simulink model "TransformerB_v4"  (R2023a)
settings: Solver=ode23tb  StartTime=0.0  StopTime=1  MaxStep=1e-4  RelTol=1e-3  EnableMultiTasking=on
undefined symbols (not defined in the file or in its folder): D11, Delta
libraries: spsSeriesRLCBranchLib x18, spsGroundLib x9, spsSaturableTransformerLib x6, spsCurrentMeasurementLib x6, spsThreePhaseFaultLib x6, spsRMSLib x6, dspstat3 x5, spsACVoltageSourceLib x3, spsThreePhaseVIMeasurementLib x2, spsThreePhaseBreakerLib x2, simulink_extras x1, simulink x1
settings Model: Creator=Admin  LastModifiedBy=Abeer
settings DataIOCC: LimitDataPoints=on  SaveFormat=Array
settings OptimizationCC: LifeSpan=inf
settings DebuggingCC: AlgebraicLoopMsg=none  SolverPrmCheckMsg=warning  SFUnexpectedBacktrackingDiag=warning  SFNoUnconditionalDefaultTransitionDiag=warning  SFExecutionAtInitializationDiag=none  ArithmeticOperatorsInVariantConditions=warning
settings HardwareCC: ProdBitPerPointer=32  ProdBitPerSizeT=32  ProdBitPerPtrDiffT=32  ProdLargestAtomicFloat=None  ProdIntDivRoundTo=Undefined  ProdEndianess=Unspecified  ProdWordSize=32  ProdHWDeviceType=32-bit Generic
settings ModelReferenceCC: PropagateSignalLabelsOutOfModel=off
settings SFSimCC: SimUseLocalCustomCode=off  CustomCodeUndefinedFunction=UseInterfaceOnly
settings RTWCC: RTWUseLocalCustomCode=off
settings CodeAppCC: StateflowObjectComments=on
settings GRTTargetCC: TargetLangStandard=C89/C90 (ANSI)
settings ConfigComp: CovMetricSettings=dw  CovSaveCumulativeToWorkspaceVar=on  CovSaveSingleToWorkspaceVar=on  CovExternalEMLEnable=off  CovSFcnEnable=off
settings SimscapeCC: SimscapeNormalizeSystem=off

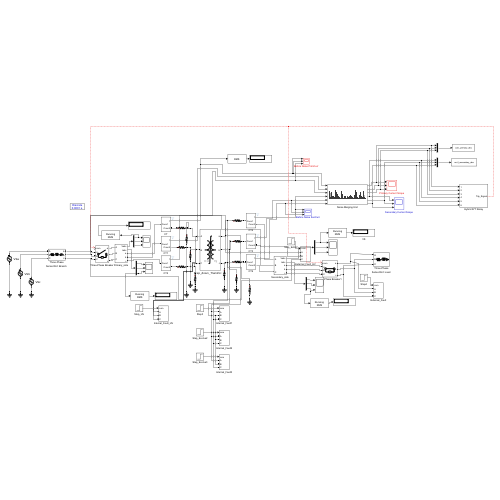
[thumbnail: Simulink's stored preview of the top-level diagram]
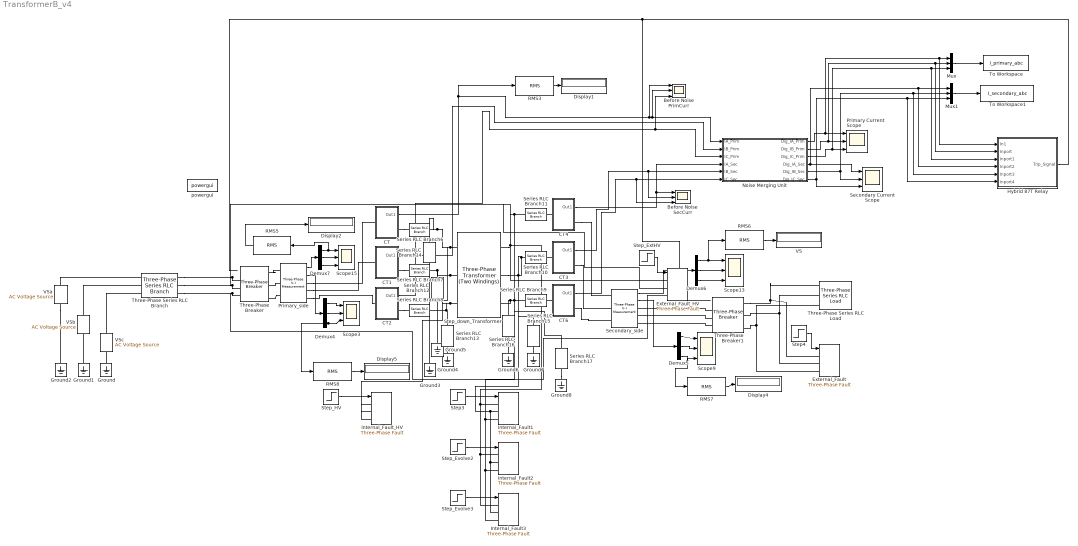
== system TransformerB_v4 ==
  Before Noise PrimCurr : Scope  NumInputPorts=3
  Before Noise SecCurr : Scope  NumInputPorts=3
  CT : Subsystem
  CT1 : Subsystem
  CT2 : Subsystem
  CT3 : Subsystem
  CT4 : Subsystem
  CT6 : Subsystem
  Demux{4..7} (4 alike) : Demux  Outputs=3
  Display{1..2,4..5} (4 alike) : Display
  External_Fault : spsThreePhaseFaultLib/Three-Phase Fault  InitialStates=0  FaultA=off  FaultB=off  FaultC=off  GroundFault=off  SwitchTimes=[0.05 1]  External=on  SwitchStatus=NaN  FaultResistance=0.001  GroundResistance=0.001  SnubberResistance=1e6  SnubberCapacitance=inf  Measurements=None
  External_Fault_HV : spsThreePhaseFaultLib/Three-Phase Fault  InitialStates=0  FaultA=off  FaultB=off  FaultC=off  GroundFault=off  SwitchTimes=[0.05 1]  External=on  SwitchStatus=NaN  FaultResistance=0.01  GroundResistance=0.01  SnubberResistance=1e6  SnubberCapacitance=inf  Measurements=None
  Ground{,1..8} (9 alike) : spsGroundLib/Ground  LConnTagsString=a
  Hybrid 87T Relay : Subsystem
  Internal_Fault1 : spsThreePhaseFaultLib/Three-Phase Fault  InitialStates=0  FaultA=off  FaultB=off  FaultC=off  GroundFault=off  SwitchTimes=[0.05 1]  External=on  SwitchStatus=NaN  FaultResistance=0.1  GroundResistance=0.01  SnubberResistance=1e6  SnubberCapacitance=inf  Measurements=None
  Internal_Fault2 : spsThreePhaseFaultLib/Three-Phase Fault  InitialStates=0  FaultA=off  FaultB=off  FaultC=off  GroundFault=off  SwitchTimes=[0.05 1]  External=on  SwitchStatus=NaN  FaultResistance=0.01  GroundResistance=0.01  SnubberResistance=1e6  SnubberCapacitance=inf  Measurements=None
  Internal_Fault3 : spsThreePhaseFaultLib/Three-Phase Fault  InitialStates=0  FaultA=off  FaultB=off  FaultC=off  GroundFault=off  SwitchTimes=[0.05 1]  External=on  SwitchStatus=NaN  FaultResistance=0.01  GroundResistance=0.01  SnubberResistance=1e6  SnubberCapacitance=inf  Measurements=None
  Internal_Fault_HV : spsThreePhaseFaultLib/Three-Phase Fault  InitialStates=0  FaultA=off  FaultB=off  FaultC=off  GroundFault=off  SwitchTimes=[0.05 1]  External=on  SwitchStatus=NaN  FaultResistance=0.01  GroundResistance=0.01  SnubberResistance=1e6  SnubberCapacitance=inf  Measurements=None
  Mux : Mux  Inputs=3
  Mux1 : Mux  Inputs=3
  Noise Merging Unit : Subsystem
      mask Display: image('$imagefile'); % Use "Edit Image" on toolstrip to change.
  Primary Current Scope : Scope  NumInputPorts=3
  Primary_side : spsThreePhaseVIMeasurementLib/Three-Phase V-I Measurement  VoltageMeasurement=phase-to-phase  SetLabelV=off  LabelV=Vabc  Vpu=off  VpuLL=off  CurrentMeasurement=yes  SetLabelI=off  LabelI=Iabc  Ipu=off  Pbase=100e6  Vbase=500e3  OutputType=Complex  PhasorSimulation=off  PSBequivalent=0
  RMS3 : dspstat3/RMS  run=off  directionMode=Each column  dimension=1  InputProcessing=Columns as channels (frame based)  reset_popup=None
  RMS{5..8} (4 alike) : dspstat3/RMS  run=on  directionMode=Each column  dimension=1  InputProcessing=Columns as channels (frame based)  reset_popup=None
  Scope{3,9,13,15} (4 alike) : Scope  NumInputPorts=3
  Secondary Current Scope : Scope  NumInputPorts=3
  Secondary_side : spsThreePhaseVIMeasurementLib/Three-Phase V-I Measurement  VoltageMeasurement=phase-to-phase  SetLabelV=off  LabelV=Vabc  Vpu=off  VpuLL=off  CurrentMeasurement=yes  SetLabelI=off  LabelI=Iabc  Ipu=off  Pbase=100e6  Vbase=500e3  OutputType=Complex  PhasorSimulation=off  PSBequivalent=0
  Series RLC Branch{6..11} (6 alike) : spsSeriesRLCBranchLib/Series RLC Branch  LConnTagsString=__new0  RConnTagsString=__new0  BranchType=R  Resistance=0.001  Inductance=1e-3  SetiL0=off  InitialCurrent=0  Capacitance=1e-6  Setx0=off  InitialVoltage=0  Measurements=None
  Series RLC Branch{12..17} (6 alike) : spsSeriesRLCBranchLib/Series RLC Branch  LConnTagsString=__new0  RConnTagsString=__new0  BranchType=C  Resistance=0.5  Inductance=1e-3  SetiL0=off  InitialCurrent=0  Capacitance=1e-9  Setx0=off  InitialVoltage=0  Measurements=None
  Step3 : Step  Time=10  SampleTime=0
  Step4 : Step  Time=0.3  SampleTime=0
  Step_Evolve2 : Step  Time=0.05  SampleTime=0
  Step_Evolve3 : Step  Time=0.05  SampleTime=0
  Step_ExtHV : Step  Time=10  SampleTime=0
  Step_HV : Step  Time=10  SampleTime=0
  Step_down_Transformer : spsThreePhaseTransformerTwoWindingsLib/Three-Phase Transformer (Two Windings)  Winding1Connection=Delta (D11)  Winding2Connection=Yg  CoreType=Three single-phase transformers  SetSaturation=on  Hysteresis=off  DataFile='hysteresis'  SetInitialFlux=off  Measurements=Winding voltages  UNITS=pu  NominalPower=[ 40e6 50 ]  Winding1=[ 132e3 0.002 0.0050 ]  Winding2=[ 33e3 0.002 0.0050 ]  Rm=500  Lm=inf  L0=0.5  Saturation=[0 0 ; 0.005 1.2 ; 5.0 1.8]  InitialFluxes=[0.8, -0.4, -0.4]  BreakLoop=off  DiscreteSolver=Trapezoidal iterative  DataType=off  TransfoNumber=1
  "Three-Phase Series RLC Branch " : spsThreePhaseSeriesRLCBranchLib/Three-Phase Series RLC Branch  LConnTagsString=A|B|C  RConnTagsString=A|B|C  BranchType=RLC  Resistance=0.46  Inductance=0.0221  Capacitance=inf  Measurements=None
  "Three-Phase Series RLC Load " : spsThreePhaseSeriesRLCLoadLib/Three-Phase Series RLC Load  LConnTagsString=A|B|C  Configuration=Y (grounded)  NominalVoltage=33e3  Vabc=[1e3 1e3 1e3]  Vabcp=[1e3 1e3 1e3]  NominalFrequency=50  UnbalancedPower=off  ActivePower=38e6  InductivePower=12.49e6  CapacitivePower=0  Pabc=[10e3 9e3 11e3]  QLabc=[100 90 110]  QCabc=[100 90 110]  Pabcp=[10e3 9e3 11e3]  QLabcp=[100 90 110]  QCabcp=[100 90 110]  Measurements=None  LoadType=constant Z
  "Three-Phase Breaker " : spsThreePhaseBreakerLib/Three-Phase Breaker  InitialState=open  SwitchA=on  SwitchB=on  SwitchC=on  SwitchTimes=[]  External=on  BreakerResistance=0.01  SnubberResistance=1e6  SnubberCapacitance=inf  Measurements=Breaker voltages and currents
  "Three-Phase Breaker1 " : spsThreePhaseBreakerLib/Three-Phase Breaker  InitialState=closed  SwitchA=on  SwitchB=on  SwitchC=on  SwitchTimes=[]  External=on  BreakerResistance=0.01  SnubberResistance=1e6  SnubberCapacitance=inf  Measurements=None
  To Workspace : ToWorkspace  VariableName=I_primary_abc  SampleTime=6.25e-4
  To Workspace1 : ToWorkspace  VariableName=I_secondary_abc  SampleTime=6.25e-4
  VS : Display
  VSa : spsACVoltageSourceLib/AC Voltage Source  Amplitude=(132e3*sqrt(2))/(sqrt(3))  Phase=0  Frequency=50  SampleTime=0  Measurements=None  BusType=swing  Pref=10e3  Qref=0  Qmin=-inf  Qmax=+inf
  VSb : spsACVoltageSourceLib/AC Voltage Source  Amplitude=(132e3*sqrt(2))/(sqrt(3))  Phase=-120  Frequency=50  SampleTime=0  Measurements=None  BusType=swing  Pref=10e3  Qref=0  Qmin=-inf  Qmax=+inf
  VSc : spsACVoltageSourceLib/AC Voltage Source  Amplitude=(132e3*sqrt(2))/(sqrt(3))  Phase=120  Frequency=50  SampleTime=0  Measurements=None  BusType=swing  Pref=10e3  Qref=0  Qmin=-inf  Qmax=+inf
  powergui : spspowerguiLib/powergui  SimulationMode=Discrete  SampleTime=10e-5  frequency=60  Iterations=50  frequencyindice=50  Pbase=100e6  ErrMax=1e-4  UnitsV=kV  UnitsW=MW  buscounter=0  FunctionMessages=off  echomessages=off  EnableUseOfTLC=off  CurrentSourceSwitches=off  DisableSnubberDevices=off  DisableRonSwitches=off  DisableVfSwitches=off  DisplayEquations=off  AutomaticDiscreteSolvers=off  SolverType=Backward Euler  Interpol=off  ExternalGateDelay=off  methode=off  Ts=0  x0status=blocks  SPID=off  SwTol=0  HookPort=off  NonlinearTolerance=1e-4  nMaxIteration=100  ContinueOnMaxIteration=off  RestoreLinks=warning  ResistiveCurrentMeasurement=off  Frange=[0:2:500]  Ylog=off  Xlog=on  ShowGrid=off  save=off  variable=ZData  structure=0  ZoomFFT=on  StartTime=0.0  cycles=1  DisplayStyle=1  fundamental=60  FreqAxis=off  MaxFrequency=1000  frequencyindicesteady=1  RmsSteady=1  display=off
  wires:
  CT/1(Out1) -> RMS3/1, Before Noise PrimCurr/1, Before Noise PrimCurr/2, Noise Merging Unit/1(IA_Prim)
  CT1/1(Out1) -> Noise Merging Unit/2(IB_Prim)
  CT2/1(Out1) -> Before Noise PrimCurr/3, Noise Merging Unit/3(IC_Prim)
  RMS3/1 -> Display1/1
  Secondary_side/2 -> Demux5/1
  Secondary_side/1 -> Demux6/1
  Demux6/1 -> RMS6/1, Scope13/1
  Demux6/2 -> Scope13/2
  Demux6/3 -> Scope13/3
  Primary_side/1 -> Demux7/1
  RMS6/1 -> VS/1
  Demux7/1 -> RMS5/1, Scope15/1
  Demux7/2 -> Scope15/2
  Demux7/3 -> Scope15/3
  RMS5/1 -> Display2/1
  Primary_side/2 -> Demux4/1
  Demux4/1 -> Scope3/1
  Demux4/2 -> Scope3/2
  Demux4/3 -> Scope3/3, RMS8/1
  RMS8/1 -> Display5/1
  CT4/1(Out1) -> Noise Merging Unit/4(IA_Sec), Before Noise SecCurr/1
  CT3/1(Out1) -> Before Noise SecCurr/2, Noise Merging Unit/5(IB_Sec)
  CT6/1(Out1) -> Before Noise SecCurr/3, Noise Merging Unit/6(IC_Sec)
  Step4/1 -> External_Fault/1
  Demux5/1 -> Scope9/1
  Demux5/2 -> Scope9/2
  Demux5/3 -> RMS7/1, Scope9/3
  RMS7/1 -> Display4/1
  Step3/1 -> Internal_Fault1/1
  Noise Merging Unit/2(Dig_IB_Prim) -> Hybrid 87T Relay/2(Inport), Mux/2, Primary Current Scope/2
  Noise Merging Unit/1(Dig_IA_Prim) -> Hybrid 87T Relay/1(In1), Mux/1, Primary Current Scope/1
  Noise Merging Unit/3(Dig_IC_Prim) -> Hybrid 87T Relay/3(Inport1), Mux/3, Primary Current Scope/3
  Noise Merging Unit/4(Dig_IA_Sec) -> Hybrid 87T Relay/4(Inport2), Mux1/1, Secondary Current Scope/1
  Noise Merging Unit/5(Dig_IB_Sec) -> Hybrid 87T Relay/5(Inport3), Mux1/2, Secondary Current Scope/2
  Noise Merging Unit/6(Dig_IC_Sec) -> Hybrid 87T Relay/6(Inport4), Mux1/3, Secondary Current Scope/3
  Mux/1 -> To Workspace/1
  Mux1/1 -> To Workspace1/1
  Hybrid 87T Relay/1(Trip_Signal) -> ?
  Step_Evolve2/1 -> Internal_Fault2/1
  Step_Evolve3/1 -> Internal_Fault3/1
  Step_HV/1 -> Internal_Fault_HV/1
  Step_ExtHV/1 -> External_Fault_HV/1
  connections:
  VSa/LConn1 -- Ground2/LConn1
  Ground/LConn1 -- VSc/LConn1
  "Three-Phase Breaker1 "/LConn1 -- Secondary_side/RConn1
  "Three-Phase Breaker1 "/LConn3 -- Secondary_side/RConn3
  "Three-Phase Breaker1 "/LConn2 -- Secondary_side/RConn2
  Ground1/LConn1 -- VSb/LConn1
  "Three-Phase Breaker "/RConn1 -- Primary_side/LConn1
  "Three-Phase Breaker "/RConn2 -- Primary_side/LConn2
  "Three-Phase Breaker "/RConn3 -- Primary_side/LConn3
  "Three-Phase Breaker1 "/RConn1 -- "Three-Phase Series RLC Load "/LConn1 -- External_Fault/LConn1
  "Three-Phase Breaker1 "/RConn2 -- "Three-Phase Series RLC Load "/LConn2 -- External_Fault/LConn2
  "Three-Phase Breaker1 "/RConn3 -- External_Fault/LConn3 -- "Three-Phase Series RLC Load "/LConn3
  Series RLC Branch6/RConn1 -- Step_down_Transformer/LConn1 -- Internal_Fault_HV/LConn1 -- Series RLC Branch14/LConn1
  CT1/RConn1 -- Series RLC Branch7/LConn1
  CT2/RConn1 -- Series RLC Branch8/LConn1
  Step_down_Transformer/RConn1 -- Internal_Fault3/LConn1 -- Internal_Fault2/LConn1 -- Internal_Fault1/LConn1 -- Series RLC Branch11/LConn1 -- Series RLC Branch17/LConn1
  Step_down_Transformer/RConn2 -- Internal_Fault3/LConn2 -- Internal_Fault2/LConn2 -- Internal_Fault1/LConn2 -- Series RLC Branch10/LConn1 -- Series RLC Branch15/LConn1
  Step_down_Transformer/RConn3 -- Internal_Fault3/LConn3 -- Internal_Fault2/LConn3 -- Internal_Fault1/LConn3 -- Series RLC Branch9/LConn1 -- Series RLC Branch16/LConn1
  "Three-Phase Breaker "/LConn1 -- "Three-Phase Series RLC Branch "/RConn1 -- External_Fault_HV/LConn1
  "Three-Phase Breaker "/LConn2 -- "Three-Phase Series RLC Branch "/RConn2 -- External_Fault_HV/LConn2
  "Three-Phase Breaker "/LConn3 -- "Three-Phase Series RLC Branch "/RConn3 -- External_Fault_HV/LConn3
  VSa/RConn1 -- "Three-Phase Series RLC Branch "/LConn1
  VSb/RConn1 -- "Three-Phase Series RLC Branch "/LConn2
  VSc/RConn1 -- "Three-Phase Series RLC Branch "/LConn3
  CT/RConn1 -- Series RLC Branch6/LConn1
  Series RLC Branch7/RConn1 -- Series RLC Branch12/LConn1 -- Step_down_Transformer/LConn2 -- Internal_Fault_HV/LConn2
  Series RLC Branch8/RConn1 -- Series RLC Branch13/LConn1 -- Step_down_Transformer/LConn3 -- Internal_Fault_HV/LConn3
  Series RLC Branch9/RConn1 -- CT6/LConn1
  Series RLC Branch10/RConn1 -- CT3/LConn1
  Series RLC Branch11/RConn1 -- CT4/LConn1
  Series RLC Branch14/RConn1 -- Ground3/LConn1
  Ground4/LConn1 -- Series RLC Branch13/RConn1
  Ground5/LConn1 -- Series RLC Branch12/RConn1
  Ground7/LConn1 -- Series RLC Branch15/RConn1
  Ground6/LConn1 -- Series RLC Branch16/RConn1
  Series RLC Branch17/RConn1 -- Ground8/LConn1
  Primary_side/RConn1 -- CT/LConn1
  Primary_side/RConn2 -- CT1/LConn1
  Primary_side/RConn3 -- CT2/LConn1
  CT4/RConn1 -- Secondary_side/LConn1
  CT3/RConn1 -- Secondary_side/LConn2
  CT6/RConn1 -- Secondary_side/LConn3

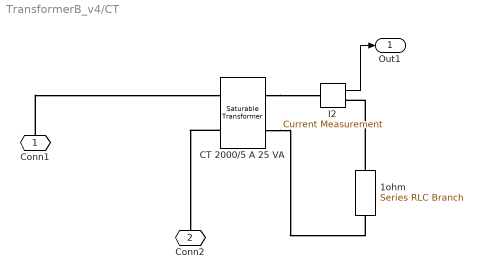
== system TransformerB_v4/CT ==
  1ohm : spsSeriesRLCBranchLib/Series RLC Branch  LConnTagsString=__new0  RConnTagsString=__new0  BranchType=R  Resistance=2.5  Inductance=[]  SetiL0=off  InitialCurrent=0  Capacitance=[]  Setx0=off  InitialVoltage=0  Measurements=None
  CT 2000/5 A 25 VA : spsSaturableTransformerLib/Saturable Transformer  ThreeWindings=off  Hysteresis=off  DataFile='hysteresis'  Measurements=Flux and magnetization current ( Imag )  UNITS=pu  NominalPower=[2.5 50]  Winding1=[2.5*(1/200) 0.05 0.001]  Winding2=[2.5 0.05 0.001]  Winding3=[5 0.001 0.04 ]  Saturation=[0 0 ; 0.001 0.8 ; 0.01 1.15 ; 0.1 1.25 ; 1 1.3]  CoreLoss=[100]  BreakLoop=off  DiscreteSolver=Trapezoidal iterative  DataType=off  InitialFlux=-4.4292901831583e-09  TransfoNumber=1
      settings: AttributesFormatString=\n  LibrarySourceBlock=sps_lib/Power Grid Elements/Saturable Transformer
  I2 : spsCurrentMeasurementLib/Current Measurement  Tag=PoWeRsYsTeMmEaSuReMeNt  PhasorSimulation=off  OutputType=Magnitude  PSBequivalent=0
      settings: AttributesFormatString=\n
  Conn1 : PMIOPort  Side=Left
  Conn2 : PMIOPort  Port=2  Side=Right
  Out1 : Outport
  wires:
  I2/1 -> Out1/1
  connections:
  CT 2000/5 A 25 VA/RConn1 -- I2/LConn1
  CT 2000/5 A 25 VA/RConn2 -- 1ohm/RConn1
  1ohm/LConn1 -- I2/RConn1
  CT 2000/5 A 25 VA/LConn2 -- Conn2/RConn1
  Conn1/RConn1 -- CT 2000/5 A 25 VA/LConn1

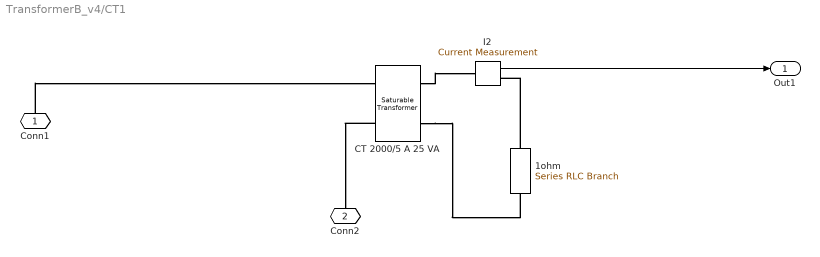
== system TransformerB_v4/CT1 ==
  1ohm : spsSeriesRLCBranchLib/Series RLC Branch  LConnTagsString=__new0  RConnTagsString=__new0  BranchType=R  Resistance=2.5  Inductance=[]  SetiL0=off  InitialCurrent=0  Capacitance=[]  Setx0=off  InitialVoltage=0  Measurements=None
  CT 2000/5 A 25 VA : spsSaturableTransformerLib/Saturable Transformer  ThreeWindings=off  Hysteresis=off  DataFile='hysteresis'  Measurements=Flux and magnetization current ( Imag )  UNITS=pu  NominalPower=[2.5 50]  Winding1=[2.5*(1/200) 0.05 0.001]  Winding2=[2.5 0.05 0.001]  Winding3=[5 0.001 0.04 ]  Saturation=[0 0 ; 0.001 0.8 ; 0.01 1.15 ; 0.1 1.25 ; 1 1.3]  CoreLoss=[100]  BreakLoop=off  DiscreteSolver=Trapezoidal iterative  DataType=off  InitialFlux=2.21150229354582e-09  TransfoNumber=1
      settings: AttributesFormatString=\n  LibrarySourceBlock=sps_lib/Power Grid Elements/Saturable Transformer
  I2 : spsCurrentMeasurementLib/Current Measurement  Tag=PoWeRsYsTeMmEaSuReMeNt  PhasorSimulation=off  OutputType=Magnitude  PSBequivalent=0
      settings: AttributesFormatString=\n
  Conn1 : PMIOPort  Side=Left
  Conn2 : PMIOPort  Port=2  Side=Right
  Out1 : Outport
  wires:
  I2/1 -> Out1/1
  connections:
  Conn1/RConn1 -- CT 2000/5 A 25 VA/LConn1
  CT 2000/5 A 25 VA/LConn2 -- Conn2/RConn1
  1ohm/LConn1 -- I2/RConn1
  CT 2000/5 A 25 VA/RConn2 -- 1ohm/RConn1
  CT 2000/5 A 25 VA/RConn1 -- I2/LConn1

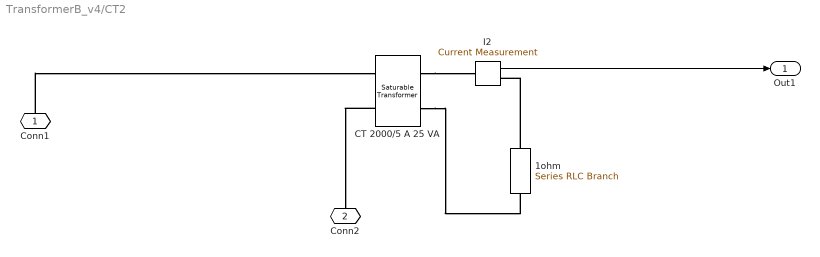
== system TransformerB_v4/CT2 ==
  1ohm : spsSeriesRLCBranchLib/Series RLC Branch  LConnTagsString=__new0  RConnTagsString=__new0  BranchType=R  Resistance=2.5  Inductance=[]  SetiL0=off  InitialCurrent=0  Capacitance=[]  Setx0=off  InitialVoltage=0  Measurements=None
  CT 2000/5 A 25 VA : spsSaturableTransformerLib/Saturable Transformer  ThreeWindings=off  Hysteresis=off  DataFile='hysteresis'  Measurements=Flux and magnetization current ( Imag )  UNITS=pu  NominalPower=[2.5 50]  Winding1=[2.5*(1/200) 0.05 0.001]  Winding2=[2.5 0.05 0.001]  Winding3=[5 0.001 0.04 ]  Saturation=[0 0 ; 0.001 0.8 ; 0.01 1.15 ; 0.1 1.25 ; 1 1.3]  CoreLoss=[100]  BreakLoop=off  DiscreteSolver=Trapezoidal iterative  DataType=off  InitialFlux=2.21778788961252e-09  TransfoNumber=1
      settings: AttributesFormatString=\n  LibrarySourceBlock=sps_lib/Power Grid Elements/Saturable Transformer
  I2 : spsCurrentMeasurementLib/Current Measurement  Tag=PoWeRsYsTeMmEaSuReMeNt  PhasorSimulation=off  OutputType=Magnitude  PSBequivalent=0
      settings: AttributesFormatString=\n
  Conn1 : PMIOPort  Side=Left
  Conn2 : PMIOPort  Port=2  Side=Right
  Out1 : Outport
  wires:
  I2/1 -> Out1/1
  connections:
  CT 2000/5 A 25 VA/RConn1 -- I2/LConn1
  CT 2000/5 A 25 VA/RConn2 -- 1ohm/RConn1
  1ohm/LConn1 -- I2/RConn1
  CT 2000/5 A 25 VA/LConn2 -- Conn2/RConn1
  Conn1/RConn1 -- CT 2000/5 A 25 VA/LConn1

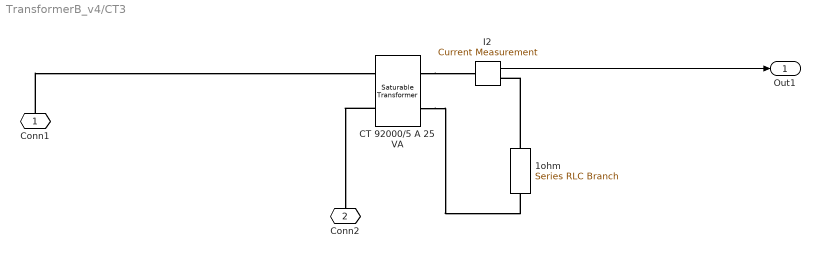
== system TransformerB_v4/CT3 ==
  1ohm : spsSeriesRLCBranchLib/Series RLC Branch  LConnTagsString=__new0  RConnTagsString=__new0  BranchType=R  Resistance=2.5  Inductance=[]  SetiL0=off  InitialCurrent=0  Capacitance=[]  Setx0=off  InitialVoltage=0  Measurements=None
  CT 92000/5 A 25 VA : spsSaturableTransformerLib/Saturable Transformer  ThreeWindings=off  Hysteresis=off  DataFile='hysteresis'  Measurements=Flux and magnetization current ( Imag )  UNITS=pu  NominalPower=[2.5 50]  Winding1=[2.5*(1/800) 0.05 0.001]  Winding2=[2.5 0.05 0.001]  Winding3=[5 0.001 0.04 ]  Saturation=[0 0 ; 0.001 0.8 ; 0.01 1.15 ; 0.1 1.25 ; 1 1.3]  CoreLoss=[100]  BreakLoop=off  DiscreteSolver=Trapezoidal iterative  DataType=off  InitialFlux=1.82966643691712e-10  TransfoNumber=1
      settings: AttributesFormatString=\n  LibrarySourceBlock=sps_lib/Power Grid Elements/Saturable Transformer
  I2 : spsCurrentMeasurementLib/Current Measurement  Tag=PoWeRsYsTeMmEaSuReMeNt  PhasorSimulation=off  OutputType=Magnitude  PSBequivalent=0
      settings: AttributesFormatString=\n
  Conn1 : PMIOPort  Side=Left
  Conn2 : PMIOPort  Port=2  Side=Right
  Out1 : Outport
  wires:
  I2/1 -> Out1/1
  connections:
  Conn1/RConn1 -- CT 92000/5 A 25 VA/LConn1
  CT 92000/5 A 25 VA/LConn2 -- Conn2/RConn1
  1ohm/LConn1 -- I2/RConn1
  CT 92000/5 A 25 VA/RConn2 -- 1ohm/RConn1
  CT 92000/5 A 25 VA/RConn1 -- I2/LConn1

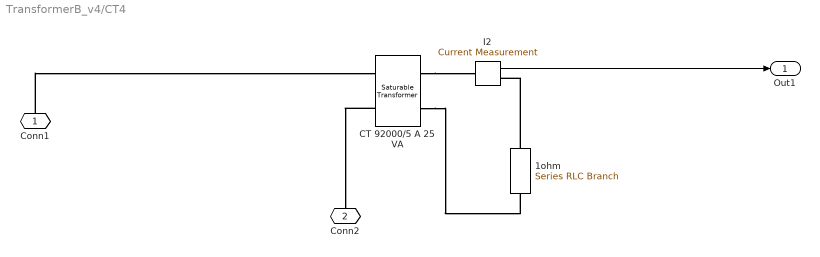
== system TransformerB_v4/CT4 ==
  1ohm : spsSeriesRLCBranchLib/Series RLC Branch  LConnTagsString=__new0  RConnTagsString=__new0  BranchType=R  Resistance=2.5  Inductance=[]  SetiL0=off  InitialCurrent=0  Capacitance=[]  Setx0=off  InitialVoltage=0  Measurements=None
  CT 92000/5 A 25 VA : spsSaturableTransformerLib/Saturable Transformer  ThreeWindings=off  Hysteresis=off  DataFile='hysteresis'  Measurements=Flux and magnetization current ( Imag )  UNITS=pu  NominalPower=[2.5 50]  Winding1=[2.5*(1/800) 0.05 0.001]  Winding2=[2.5 0.05 0.001]  Winding3=[5 0.001 0.04 ]  Saturation=[0 0 ; 0.001 0.8 ; 0.01 1.15 ; 0.1 1.25 ; 1 1.3]  CoreLoss=[100]  BreakLoop=off  DiscreteSolver=Trapezoidal iterative  DataType=off  InitialFlux=-1.83122766517186e-10  TransfoNumber=1
      settings: AttributesFormatString=\n  LibrarySourceBlock=sps_lib/Power Grid Elements/Saturable Transformer
  I2 : spsCurrentMeasurementLib/Current Measurement  Tag=PoWeRsYsTeMmEaSuReMeNt  PhasorSimulation=off  OutputType=Magnitude  PSBequivalent=0
      settings: AttributesFormatString=\n
  Conn1 : PMIOPort  Side=Left
  Conn2 : PMIOPort  Port=2  Side=Right
  Out1 : Outport
  wires:
  I2/1 -> Out1/1
  connections:
  CT 92000/5 A 25 VA/RConn1 -- I2/LConn1
  CT 92000/5 A 25 VA/RConn2 -- 1ohm/RConn1
  1ohm/LConn1 -- I2/RConn1
  CT 92000/5 A 25 VA/LConn2 -- Conn2/RConn1
  Conn1/RConn1 -- CT 92000/5 A 25 VA/LConn1

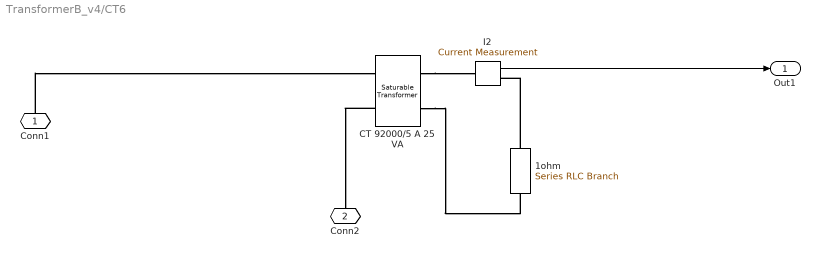
== system TransformerB_v4/CT6 ==
  1ohm : spsSeriesRLCBranchLib/Series RLC Branch  LConnTagsString=__new0  RConnTagsString=__new0  BranchType=R  Resistance=2.5  Inductance=[]  SetiL0=off  InitialCurrent=0  Capacitance=[]  Setx0=off  InitialVoltage=0  Measurements=None
  CT 92000/5 A 25 VA : spsSaturableTransformerLib/Saturable Transformer  ThreeWindings=off  Hysteresis=off  DataFile='hysteresis'  Measurements=Flux and magnetization current ( Imag )  UNITS=pu  NominalPower=[2.5 50]  Winding1=[2.5*(1/800) 0.05 0.001]  Winding2=[2.5 0.05 0.001]  Winding3=[5 0.001 0.04 ]  Saturation=[0 0 ; 0.001 0.8 ; 0.01 1.15 ; 0.1 1.25 ; 1 1.3]  CoreLoss=[100]  BreakLoop=off  DiscreteSolver=Trapezoidal iterative  DataType=off  InitialFlux=1.56122825475519e-13  TransfoNumber=1
      settings: AttributesFormatString=\n  LibrarySourceBlock=sps_lib/Power Grid Elements/Saturable Transformer
  I2 : spsCurrentMeasurementLib/Current Measurement  Tag=PoWeRsYsTeMmEaSuReMeNt  PhasorSimulation=off  OutputType=Magnitude  PSBequivalent=0
      settings: AttributesFormatString=\n
  Conn1 : PMIOPort  Side=Left
  Conn2 : PMIOPort  Port=2  Side=Right
  Out1 : Outport
  wires:
  I2/1 -> Out1/1
  connections:
  CT 92000/5 A 25 VA/RConn1 -- I2/LConn1
  CT 92000/5 A 25 VA/RConn2 -- 1ohm/RConn1
  1ohm/LConn1 -- I2/RConn1
  CT 92000/5 A 25 VA/LConn2 -- Conn2/RConn1
  Conn1/RConn1 -- CT 92000/5 A 25 VA/LConn1

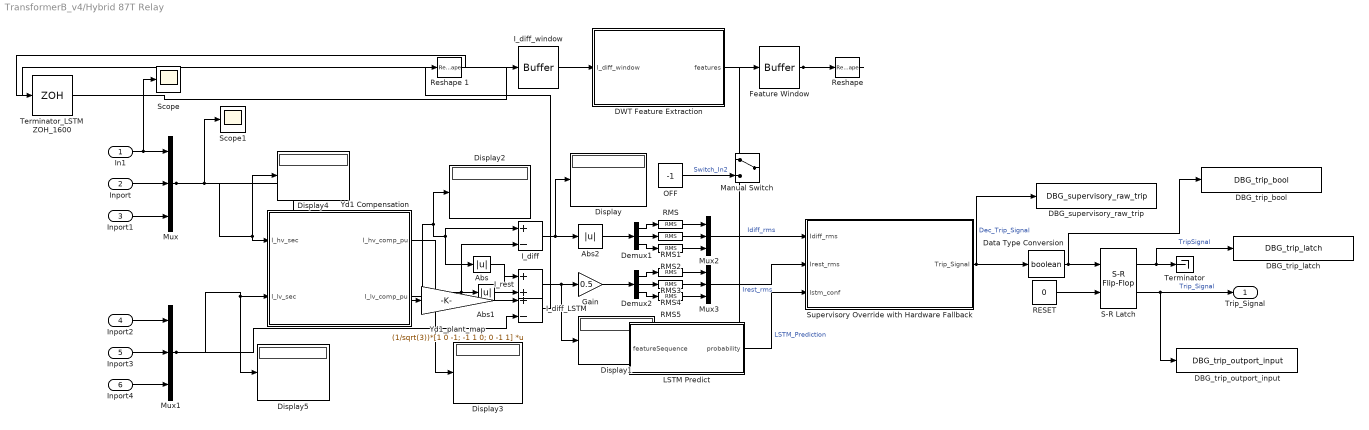
== system TransformerB_v4/Hybrid 87T Relay ==
  In1 : Inport
  Inport : Inport  Port=2
  Inport1 : Inport  Port=3
  Inport2 : Inport  Port=4
  Inport3 : Inport  Port=5
  Inport4 : Inport  Port=6
  Abs : Abs  SaturateOnIntegerOverflow=off
  Abs1 : Abs  SaturateOnIntegerOverflow=off
  Abs2 : Abs  SaturateOnIntegerOverflow=off
  DBG_supervisory_raw_trip : ToWorkspace  VariableName=DBG_supervisory_raw_trip  SampleTime=-1
  DBG_trip_bool : ToWorkspace  VariableName=DBG_trip_bool  SampleTime=-1
  DBG_trip_latch : ToWorkspace  VariableName=DBG_trip_latch  SampleTime=-1
  DBG_trip_outport_input : ToWorkspace  VariableName=DBG_trip_outport_input  SampleTime=-1
  DWT Feature Extraction : MATLAB Function  TreatAsAtomicUnit=on
  Data Type Conversion : DataTypeConversion  OutDataTypeStr=boolean  SaturateOnIntegerOverflow=off  RndMeth=Floor
  Demux1 : Demux  Outputs=3
  Demux2 : Demux  Outputs=3
  Display{,1..5} (6 alike) : Display
  Feature Window : Buffer  N=32  V=31  OutputFrames=off
  Gain : Gain  Gain=0.5
  I_diff : Sum  Inputs=|+-
  I_diff_LSTM : Sum  Inputs=+-
  I_diff_window : Buffer  N=32  V=31  OutputFrames=off
  I_rest : Sum  Inputs=|++
  LSTM Predict : MATLAB Function  TreatAsAtomicUnit=on
  Manual Switch : ManualSwitch
  Mux{,1..3} (4 alike) : Mux  Inputs=3
  OFF : Constant  Value=-1
  RESET : Constant  Value=0  OutDataTypeStr=boolean
  RMS{,1..5} (6 alike) : spsRMSLib/RMS  TrueRMS=on  Freq=50  RMSInit=0  Ts=0.0001
  "Reshape " : Reshape  OutputDimensionality=Customize  OutputDimensions=[1, 32, 12]
  Reshape 1 : Reshape  OutputDimensionality=Customize  OutputDimensions=[1, 3]
  S-R Latch : simulink_extras/Flip Flops/S-R Flip-Flop  initial_condition=0
  Scope : Scope
  Scope1 : Scope
  Supervisory Override with Hardware Fallback : MATLAB Function  TreatAsAtomicUnit=on
  Terminator : Terminator
  Terminator_LSTM : Terminator
  Yd1 Compensation : MATLAB Function  TreatAsAtomicUnit=on
  Yd1_plant_map : Gain  Gain=(1/sqrt(3))*[1 0 -1; -1 1 0; 0 -1 1]  Multiplication=Matrix(K*u)
  ZOH_1600 : ZeroOrderHold  SampleTime=6.25e-4
  Trip_Signal : Outport
  wires:
  Inport3/1 -> Mux1/2
  Inport2/1 -> Mux1/1
  Inport4/1 -> Mux1/3
  In1/1 -> Scope/1, Mux/1
  Inport/1 -> Mux/2
  Inport1/1 -> Mux/3
  Mux/1 -> Scope1/1, Display4/1, Yd1 Compensation/1(I_hv_sec), Yd1_plant_map/1
  Mux1/1 -> Display5/1, Yd1 Compensation/2(I_lv_sec), I_diff_LSTM/2
  Yd1 Compensation/2(I_lv_comp_pu) -> Abs/1, I_diff/1, Display2/1
  Yd1 Compensation/1(I_hv_comp_pu) -> Display3/1, Abs1/1, I_diff/2
  Abs1/1 -> I_rest/2
  Abs/1 -> I_rest/1
  I_rest/1 -> Display1/1, Gain/1
  I_diff/1 -> Abs2/1, Display/1
  I_diff_window/1 -> DWT Feature Extraction/1(I_diff_window)
  DWT Feature Extraction/1(features) -> Feature Window/1
  Feature Window/1 -> "Reshape "/1, Terminator_LSTM/1
  Mux3/1 -> Supervisory Override with Hardware Fallback/2(Irest_rms)  "Irest_rms"
  Supervisory Override with Hardware Fallback/1(Trip_Signal) -> Data Type Conversion/1, DBG_supervisory_raw_trip/1  "Dec_Trip_Signal"
  OFF/1 -> Manual Switch/2  "Switch_In2"
  S-R Latch/2 -> Trip_Signal/1, DBG_trip_outport_input/1  "Trip_Signal"
  Abs2/1 -> Demux1/1
  Demux1/1 -> RMS/1
  Demux1/2 -> RMS1/1
  Demux1/3 -> RMS2/1
  Demux2/2 -> RMS4/1
  Gain/1 -> Demux2/1
  Demux2/1 -> RMS3/1
  Demux2/3 -> RMS5/1
  RMS1/1 -> Mux2/2
  RMS2/1 -> Mux2/3
  RMS/1 -> Mux2/1
  Mux2/1 -> Supervisory Override with Hardware Fallback/1(Idiff_rms)  "Idiff_rms"
  RMS3/1 -> Mux3/1
  RMS5/1 -> Mux3/3
  RMS4/1 -> Mux3/2
  RESET/1 -> S-R Latch/2
  Data Type Conversion/1 -> S-R Latch/1, DBG_trip_bool/1
  S-R Latch/1 -> DBG_trip_latch/1, Terminator/1  "TripSignal"
  I_diff_LSTM/1 -> Reshape 1/1
  Yd1_plant_map/1 -> I_diff_LSTM/1
  Reshape 1/1 -> ZOH_1600/1
  ZOH_1600/1 -> I_diff_window/1
  "Reshape "/1 -> LSTM Predict/1(featureSequence)
  LSTM Predict/1(probability) -> Supervisory Override with Hardware Fallback/3(lstm_conf)  "LSTM_Prediction"

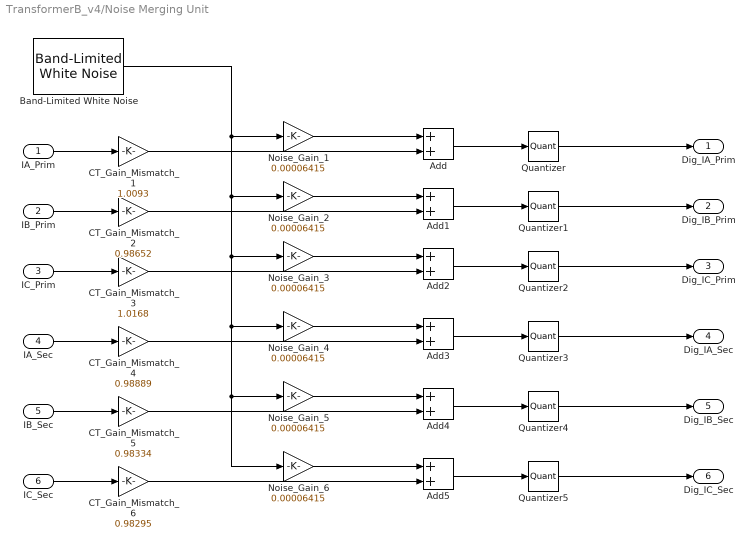
== system TransformerB_v4/Noise Merging Unit ==
  IA_Prim : Inport
  IB_Prim : Inport  Port=2
  IC_Prim : Inport  Port=3
  IA_Sec : Inport  Port=4
  IB_Sec : Inport  Port=5
  IC_Sec : Inport  Port=6
  Add{,1..5} (6 alike) : Sum
  Band-Limited White Noise : simulink/Sources/Band-Limited White Noise  Cov=[0.1]  Ts=0.0001  seed=[23341]
  CT_Gain_Mismatch_1 : Gain  Gain=1.0093
  CT_Gain_Mismatch_2 : Gain  Gain=0.98652
  CT_Gain_Mismatch_3 : Gain  Gain=1.0168
  CT_Gain_Mismatch_4 : Gain  Gain=0.98889
  CT_Gain_Mismatch_5 : Gain  Gain=0.98334
  CT_Gain_Mismatch_6 : Gain  Gain=0.98295
  Noise_Gain_{1..6} (6 alike) : Gain  Gain=0.00006415
  Quantizer{,1..5} (6 alike) : Quantizer  QuantizationInterval=0.01
  Dig_IA_Prim : Outport
  Dig_IB_Prim : Outport  Port=2
  Dig_IC_Prim : Outport  Port=3
  Dig_IA_Sec : Outport  Port=4
  Dig_IB_Sec : Outport  Port=5
  Dig_IC_Sec : Outport  Port=6
  wires:
  IA_Prim/1 -> CT_Gain_Mismatch_1/1
  IB_Prim/1 -> CT_Gain_Mismatch_2/1
  IC_Prim/1 -> CT_Gain_Mismatch_3/1
  IA_Sec/1 -> CT_Gain_Mismatch_4/1
  IB_Sec/1 -> CT_Gain_Mismatch_5/1
  IC_Sec/1 -> CT_Gain_Mismatch_6/1
  Add/1 -> Quantizer/1
  Add1/1 -> Quantizer1/1
  Add2/1 -> Quantizer2/1
  CT_Gain_Mismatch_1/1 -> Add/2
  CT_Gain_Mismatch_2/1 -> Add1/2
  CT_Gain_Mismatch_3/1 -> Add2/2
  Add3/1 -> Quantizer3/1
  CT_Gain_Mismatch_4/1 -> Add3/2
  Add4/1 -> Quantizer4/1
  CT_Gain_Mismatch_5/1 -> Add4/2
  Add5/1 -> Quantizer5/1
  CT_Gain_Mismatch_6/1 -> Add5/2
  Quantizer/1 -> Dig_IA_Prim/1
  Quantizer1/1 -> Dig_IB_Prim/1
  Quantizer2/1 -> Dig_IC_Prim/1
  Quantizer3/1 -> Dig_IA_Sec/1
  Quantizer4/1 -> Dig_IB_Sec/1
  Quantizer5/1 -> Dig_IC_Sec/1
  Band-Limited White Noise/1 -> Noise_Gain_6/1, Noise_Gain_5/1, Noise_Gain_4/1, Noise_Gain_3/1, Noise_Gain_2/1, Noise_Gain_1/1
  Noise_Gain_1/1 -> Add/1
  Noise_Gain_2/1 -> Add1/1
  Noise_Gain_3/1 -> Add2/1
  Noise_Gain_4/1 -> Add3/1
  Noise_Gain_5/1 -> Add4/1
  Noise_Gain_6/1 -> Add5/1

== matlab function TransformerB_v4/Hybrid 87T Relay/DWT Feature Extraction ==
  data: I_diff_window input; features output
function features = DWT_Feature_Extraction(I_diff_window)
    % Inputs: I_diff_window (32x3 matrix from the Buffer block)
    % Outputs: features (1x12 vector for the LSTM)
    % Step 1.4: Normalised to per-unit using rated secondary current (1.8610 A)
    
    % wavelets and fft are extrinsic because code generator does not support dwt/wavedec/fft
    coder.extrinsic('wavedec', 'detcoef', 'appcoef', 'fft');
    
    features = zeros(1, 12);
    I_base = 1.8610; % rated CT-secondary base current for v4 (probe_ct_truth_v4.m)
    
    for ph = 1:3
        signal = I_diff_window(:, ph) / I_base;
        
        % Pre-initialize variables for code generation compliance
        C = zeros(45, 1);
        L = zeros(4, 1);
        d1 = zeros(19, 1);
        d2 = zeros(13, 1);
        a2 = zeros(13, 1);
        fft_vals = zeros(32, 1);
        
        % 2-level db4 wavelet decomposition
        [C, L] = wavedec(signal, 2, 'db4');
        
        % Calculate squared DWT energy coefficients
        d1 = detcoef(C, L, 1);
        d2 = detcoef(C, L, 2);
        a2 = appcoef(C, L, 'db4', 2);
        
        E_D1 = sum(d1.^2);
        E_D2 = sum(d2.^2);
        E_A2 = sum(a2.^2);
        
        % Store features in 12-element feature vector
        base = (ph - 1) * 3 + 1;
        features(base)     = log(1 + E_D1);
        features(base + 1) = log(1 + E_D2);
        features(base + 2) = log(1 + E_A2);
        
        % 2nd Harmonic Ratio (Bin 3 = 100 Hz, Bin 2 = 50 Hz @ 1600 Hz / 32 samples)
        fft_vals = abs(fft(signal));
        ratio_2nd = fft_vals(3) / (fft_vals(2) + 1e-4);
        features(9 + ph) = min(ratio_2nd, 2.0);
    end
end

== matlab function TransformerB_v4/Hybrid 87T Relay/Yd1 Compensation ==
  data: I_hv_comp_pu output; I_hv_sec input; I_lv_comp_pu output; I_lv_sec input
function [I_hv_comp_pu, I_lv_comp_pu] = Yd1_Compensation(I_hv_sec, I_lv_sec)
% =========================================================================
% HYBRID ADAPTIVE 87T RELAY: SIGNAL CONDITIONING & COMPENSATION (Plant B)
% Vector Group: Dyn11 (HV Delta, LV Wye). 40 MVA, 132/33 kV, 1 A secondaries
% Calibrated: 2026-10-27 from probe_ct_truth_plant_b.m
% =========================================================================
    % 1. NAMEPLATE RATINGS (40 MVA)
    S_nom   = 40e6;
    V_hv_ll = 132e3;
    V_lv_ll = 33e3;

    % 2. Primary full-load amperes
    I_FLA_hv = S_nom / (sqrt(3) * V_hv_ll);   % 174.9546 A
    I_FLA_lv = S_nom / (sqrt(3) * V_lv_ll);   % 699.8184 A

    % 3. EFFECTIVE CT ratios
    CT_Ratio_HV = 202.0119;
    CT_Ratio_LV = 808.8849;

    % 4. Rated secondary currents = 1.0 pu bases (Mean: 0.8232 A)
    I_nom = 0.8232;

    % 5. Per-unit normalisation
    I_hv_pu = I_hv_sec ./ I_nom;
    I_lv_pu = I_lv_sec ./ I_nom;

    % 6. Dyn11 compensation of the Wye (LV) side.
    % M2 matrix yields 0.0353 pu residual (pure magnetizing current).
    M_Dyn11 = (1/sqrt(3)) * [ 1, -1,  0; 
                              0,  1, -1; 
                             -1,  0,  1];
    I_lv_comp_pu = M_Dyn11 * I_lv_pu;

    % HV (Delta) side passes through
    I_hv_comp_pu = I_hv_pu;
end

== matlab function TransformerB_v4/Hybrid 87T Relay/LSTM Predict ==
  data: featureSequence input; probability output
function probability = LSTM_Predict(featureSequence)
%#codegen
% Simulation-only wrapper around live_relay_ai.
coder.extrinsic('lstm_predict_wrapper');
probability = 0.0;
probability = lstm_predict_wrapper(featureSequence);
end

== matlab function TransformerB_v4/Hybrid 87T Relay/Supervisory Override with Hardware Fallback ==
  data: Idiff_rms input; Trip_Signal output; Irest_rms input; lstm_conf input
function Trip_Signal = Hybrid_87T_Decision(Idiff_rms, Irest_rms, lstm_conf)
% Inputs:
%   Idiff_rms  : 3x1 vector of differential current RMS magnitudes (p.u.)
%   Irest_rms  : 3x1 vector of restraint current RMS magnitudes (p.u.)
%   lstm_conf  : scalar, WT-LSTM confidence that the event is a FAULT (0–1)
%                Pass -1 to disable AI and fall back to pure 87T logic.
% Output:
%   Trip_Signal: 1 = Trip, 0 = Block

    % --- RELAY SETTINGS ---
    I_pickup     = 0.30;
    I_high_set   = 10.0;
    Slope_1      = 0.25;
    Slope_2      = 0.60;
    Breakpoint   = 3.0;
    AI_Threshold = 0.9900;
    AI_Solo_Threshold = 0.9980;   % option 2: AI-alone trip (no 87T vote needed)

    Trip_Signal   = 0;   % default: block
    any_87t_trip  = false;

    % --- PHASE-BY-PHASE EVALUATION ---
    for ph = 1:3
        Id = Idiff_rms(ph);
        Ir = Irest_rms(ph);

        % 1. INSTANTANEOUS OVERRIDE (catastrophic fault — no AI veto allowed)
        if Id > I_high_set
            Trip_Signal = 1;
            return;          % immediate exit, hardware speed trip
        end

        % 2. ADAPTIVE 87T LOGIC
        trip_87t = 0;
        if Id > I_pickup
            if Ir <= Breakpoint
                if Id > (Slope_1 * Ir)
                    trip_87t = 1;
                end
            else
                dynamic_bias = (Slope_2 * (Ir - Breakpoint)) + (Slope_1 * Breakpoint);
                if Id > dynamic_bias
                    trip_87t = 1;
                end
            end
        end

        % Accumulate: if ANY phase votes trip, flag it
        if trip_87t == 1
            any_87t_trip = true;
        end
    end

    % --- HYBRID AI HANDSHAKE (evaluated ONCE after all phases) ---
    % Only reached if no instantaneous override fired above.
    if any_87t_trip
        if lstm_conf == -1
            % FALLBACK MODE: AI disabled, 87T decides alone
            Trip_Signal = 1;
        elseif lstm_conf >= AI_Threshold
            % HYBRID MODE: AI confirms the fault
            Trip_Signal = 1;
        end
        % lstm_conf in [0, AI_Threshold): AI veto (inrush / CT saturation)
        % Trip_Signal stays 0
    end
    % --- AI-ALONE PATH (option 2): a very high CONFIRMED LSTM score trips without an 87T vote ---
    if Trip_Signal == 0 && lstm_conf ~= -1 && lstm_conf >= AI_Solo_Threshold
        Trip_Signal = 1;
    end

end
